simulink model "UAV_Load_Balancing_Main"  (R2025b)
settings: Solver=ode23t  StartTime=0.0  StopTime=8  FixedStep=1e-5  MaxStep=1e-5  RelTol=1e-3
libraries: nesl_utility x67, fl_lib x49, ee_lib x36
(part 2 of 2)

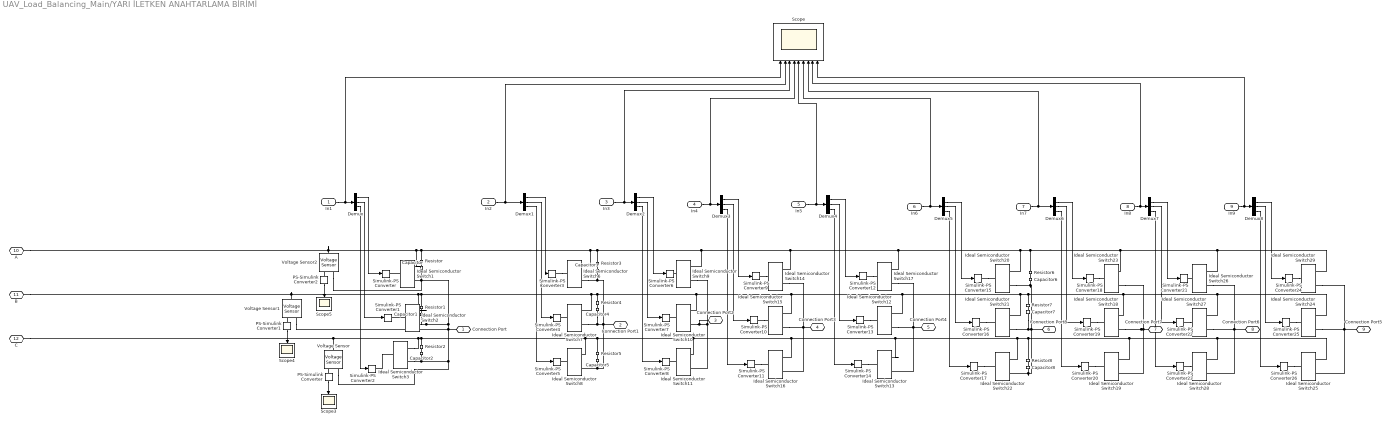
== system UAV_Load_Balancing_Main/YARI İLETKEN ANAHTARLAMA BİRİMİ ==
  In1 : Inport
  In2 : Inport  Port=2
  In3 : Inport  Port=3
  In4 : Inport  Port=4
  In5 : Inport  Port=5
  In6 : Inport  Port=6
  In7 : Inport  Port=7
  In8 : Inport  Port=8
  In9 : Inport  Port=9
  Capacitor{,3..8} (7 alike) : fl_lib/Electrical/Electrical Elements/Capacitor  c=100e-8 F  r=1e-6 Ohm  g=0 1/Ohm  i_specify=off  i_priority=None  i=0 A  i_nominal_specify=off  i_nominal_value=1  i_nominal_unit=A  v_specify=off  v_priority=None  v=0 V  v_nominal_specify=off  v_nominal_value=1  v_nominal_unit=V  vc_specify=off  vc_priority=High  vc=0 V  vc_nominal_specify=off  vc_nominal_value=1  vc_nominal_unit=V
  Capacitor1 : fl_lib/Electrical/Electrical Elements/Capacitor  c=100e-9 F  r=1e-6 Ohm  g=0 1/Ohm  i_specify=off  i_priority=None  i=0 A  i_nominal_specify=off  i_nominal_value=1  i_nominal_unit=A  v_specify=off  v_priority=None  v=0 V  v_nominal_specify=off  v_nominal_value=1  v_nominal_unit=V  vc_specify=off  vc_priority=High  vc=0 V  vc_nominal_specify=off  vc_nominal_value=1  vc_nominal_unit=V
  Capacitor2 : fl_lib/Electrical/Electrical Elements/Capacitor  c=100e-9 F  r=1e-6 Ohm  g=0 1/Ohm  i_specify=off  i_priority=None  i=0 A  i_nominal_specify=off  i_nominal_value=1  i_nominal_unit=A  v_specify=off  v_priority=None  v=0 V  v_nominal_specify=off  v_nominal_value=1  v_nominal_unit=V  vc_specify=off  vc_priority=High  vc=0 V  vc_nominal_specify=off  vc_nominal_value=1  vc_nominal_unit=V
  Demux{,1..8} (9 alike) : Demux  Outputs=3
  Ideal Semiconductor Switch{1..3,6..29} (27 alike) : ee_lib/Semiconductors & Converters/Ideal Semiconductor Switch  port_option=ee.enum.controlport.ps  Ron=0.001 Ohm  Goff=1e-6 1/Ohm  Vth=0.5 V  diode_param=ee.enum.semiconductors.protectionDiode.external  diode_Vf=0.8 V  diode_Ron=0.001 Ohm  diode_Goff=1e-5 1/Ohm  diode_C=50e-9 F  diode_iRM=-235 A  diode_iF=300 A  diode_idot=-50 A/us  diode_trr_param=ee.enum.converters.diodetrr.trr_factor  diode_trr_factor=3  diode_trr=15 us  diode_Qrr=1500 s*uA
  PS-Simulink Converter : nesl_utility/PS-Simulink Converter  PhysicalDomain=network_engine_domain  SubClassName=ps_output  LeftPortType=input  RightPortType=output  PseudoPeriodic=off  Frequencies=[]  VectorFormat=inherit  Unit=inherit  AffineConversion=off
  PS-Simulink Converter1 : nesl_utility/PS-Simulink Converter  PhysicalDomain=network_engine_domain  SubClassName=ps_output  LeftPortType=input  RightPortType=output  PseudoPeriodic=off  Frequencies=[]  VectorFormat=inherit  Unit=inherit  AffineConversion=off
  PS-Simulink Converter2 : nesl_utility/PS-Simulink Converter  PhysicalDomain=network_engine_domain  SubClassName=ps_output  LeftPortType=input  RightPortType=output  PseudoPeriodic=off  Frequencies=[]  VectorFormat=inherit  Unit=inherit  AffineConversion=off
  Resistor{,1..8} (9 alike) : fl_lib/Electrical/Electrical Elements/Resistor  R=100 Ohm  i_specify=off  i_priority=None  i=0 A  i_nominal_specify=off  i_nominal_value=1  i_nominal_unit=A  v_specify=off  v_priority=None  v=0 V  v_nominal_specify=off  v_nominal_value=1  v_nominal_unit=V
  Scope : Scope  NumInputPorts=9
      settings: ActiveDisplayYMinimum=-0.12499999999999997  ActiveDisplayYMaximum=1.125  DataLoggingVariableName=ScopeData4
  Scope3 : Scope
      settings: ActiveDisplayYMinimum=-516.00963251319388  ActiveDisplayYMaximum=519.11570917932033  DataLoggingVariableName=ScopeData9
  Scope4 : Scope
      settings: ActiveDisplayYMinimum=-401.22807276870481  ActiveDisplayYMaximum=439.38830667232617  DataLoggingVariableName=ScopeData12
  Scope5 : Scope
      settings: ActiveDisplayYMinimum=-675.65927167649568  ActiveDisplayYMaximum=614.86430923412968  DataLoggingVariableName=ScopeData13
  Simulink-PS Converter : nesl_utility/Simulink-PS Converter  PhysicalDomain=network_engine_domain  SubClassName=ps_input  LeftPortType=input  RightPortType=output  PseudoPeriodic=off  Frequencies=[]  NoiseDistribution=none  NoiseParameters=[]  Unit=V  AffineConversion=off  FilteringAndDerivatives=provide  SimscapeFilterOrder=1  InputFilterTimeConstant=0.001  UdotUserProvided=0
  Simulink-PS Converter1 : nesl_utility/Simulink-PS Converter  PhysicalDomain=network_engine_domain  SubClassName=ps_input  LeftPortType=input  RightPortType=output  PseudoPeriodic=off  Frequencies=[]  NoiseDistribution=none  NoiseParameters=[]  Unit=V  AffineConversion=off  FilteringAndDerivatives=provide  SimscapeFilterOrder=1  InputFilterTimeConstant=0.001  UdotUserProvided=0
  Simulink-PS Converter{3..26} (24 alike) : nesl_utility/Simulink-PS Converter  PhysicalDomain=network_engine_domain  SubClassName=ps_input  LeftPortType=input  RightPortType=output  PseudoPeriodic=off  Frequencies=[]  NoiseDistribution=none  NoiseParameters=[]  Unit=1  AffineConversion=off  FilteringAndDerivatives=provide  SimscapeFilterOrder=1  InputFilterTimeConstant=0.001  UdotUserProvided=0
  Simulink-PS Converter2 : nesl_utility/Simulink-PS Converter  PhysicalDomain=network_engine_domain  SubClassName=ps_input  LeftPortType=input  RightPortType=output  PseudoPeriodic=off  Frequencies=[]  NoiseDistribution=none  NoiseParameters=[]  Unit=V  AffineConversion=off  FilteringAndDerivatives=provide  SimscapeFilterOrder=1  InputFilterTimeConstant=0.001  UdotUserProvided=0
  Voltage Sensor : fl_lib/Electrical/Electrical Sensors/Voltage Sensor
  Voltage Sensor1 : fl_lib/Electrical/Electrical Sensors/Voltage Sensor
  Voltage Sensor2 : fl_lib/Electrical/Electrical Sensors/Voltage Sensor
  Connection Port : PMIOPort  Side=Right
  Connection Port1 : PMIOPort  Port=2  Side=Right
  Connection Port2 : PMIOPort  Port=3  Side=Right
  Connection Port3 : PMIOPort  Port=4  Side=Right
  Connection Port4 : PMIOPort  Port=5  Side=Right
  Connection Port8 : PMIOPort  Port=6  Side=Right
  Connection Port7 : PMIOPort  Port=7  Side=Right
  Connection Port6 : PMIOPort  Port=8  Side=Right
  Connection Port5 : PMIOPort  Port=9  Side=Right
  A : PMIOPort  Port=10  Side=Left
  B : PMIOPort  Port=11  Side=Left
  C : PMIOPort  Port=12  Side=Left
  wires:
  In1/1 -> Scope/1, Demux/1
  Demux1/3 -> Simulink-PS Converter5/1
  Demux1/1 -> Simulink-PS Converter3/1
  Demux1/2 -> Simulink-PS Converter4/1
  In2/1 -> Scope/2, Demux1/1
  Demux2/3 -> Simulink-PS Converter8/1
  Demux2/1 -> Simulink-PS Converter6/1
  Demux2/2 -> Simulink-PS Converter7/1
  In3/1 -> Scope/3, Demux2/1
  Demux3/3 -> Simulink-PS Converter11/1
  Demux3/1 -> Simulink-PS Converter9/1
  Demux3/2 -> Simulink-PS Converter10/1
  In4/1 -> Scope/4, Demux3/1
  Demux4/3 -> Simulink-PS Converter14/1
  Demux4/1 -> Simulink-PS Converter12/1
  Demux4/2 -> Simulink-PS Converter13/1
  In5/1 -> Demux4/1, Scope/5
  Demux5/3 -> Simulink-PS Converter17/1
  Demux5/1 -> Simulink-PS Converter15/1
  Demux5/2 -> Simulink-PS Converter16/1
  In6/1 -> Scope/6, Demux5/1
  Demux6/3 -> Simulink-PS Converter20/1
  Demux6/1 -> Simulink-PS Converter18/1
  Demux6/2 -> Simulink-PS Converter19/1
  In7/1 -> Scope/7, Demux6/1
  Demux7/3 -> Simulink-PS Converter23/1
  Demux7/1 -> Simulink-PS Converter21/1
  Demux7/2 -> Simulink-PS Converter22/1
  In8/1 -> Scope/8, Demux7/1
  Demux8/3 -> Simulink-PS Converter26/1
  Demux8/1 -> Simulink-PS Converter24/1
  Demux8/2 -> Simulink-PS Converter25/1
  In9/1 -> Scope/9, Demux8/1
  PS-Simulink Converter/1 -> Scope3/1
  Demux/3 -> Simulink-PS Converter2/1
  PS-Simulink Converter1/1 -> Scope4/1
  PS-Simulink Converter2/1 -> Scope5/1
  Demux/2 -> Simulink-PS Converter1/1
  Demux/1 -> Simulink-PS Converter/1
  connections:
  Connection Port/RConn1 -- Ideal Semiconductor Switch3/RConn2 -- Capacitor2/RConn1 -- Voltage Sensor/RConn2 -- Capacitor1/RConn1 -- Ideal Semiconductor Switch2/RConn2 -- Capacitor/RConn1 -- Voltage Sensor2/RConn2 -- Ideal Semiconductor Switch1/RConn2 -- Voltage Sensor1/RConn2
  B/RConn1 -- Voltage Sensor1/LConn1 -- Resistor1/LConn1 -- Ideal Semiconductor Switch7/RConn1 -- Resistor4/LConn1 -- Ideal Semiconductor Switch10/RConn1 -- Ideal Semiconductor Switch15/RConn1 -- Ideal Semiconductor Switch12/RConn1 -- Ideal Semiconductor Switch21/RConn1 -- Resistor7/LConn1 -- Ideal Semiconductor Switch18/RConn1 -- Ideal Semiconductor Switch27/RConn1 -- Ideal Semiconductor Switch24/RConn1 -- Ideal Semiconductor Switch2/RConn1
  Ideal Semiconductor Switch6/RConn2 -- Capacitor3/RConn1 -- Capacitor4/RConn1 -- Ideal Semiconductor Switch7/RConn2 -- Connection Port1/RConn1 -- Capacitor5/RConn1 -- Ideal Semiconductor Switch8/RConn2
  Ideal Semiconductor Switch29/RConn2 -- Connection Port5/RConn1 -- Ideal Semiconductor Switch24/RConn2 -- Ideal Semiconductor Switch25/RConn2
  Ideal Semiconductor Switch26/RConn2 -- Ideal Semiconductor Switch28/RConn2 -- Connection Port6/RConn1 -- Ideal Semiconductor Switch27/RConn2
  Ideal Semiconductor Switch23/RConn2 -- Ideal Semiconductor Switch18/RConn2 -- Connection Port7/RConn1 -- Ideal Semiconductor Switch19/RConn2
  Ideal Semiconductor Switch20/RConn2 -- Capacitor6/RConn1 -- Capacitor7/RConn1 -- Ideal Semiconductor Switch21/RConn2 -- Connection Port8/RConn1 -- Capacitor8/RConn1 -- Ideal Semiconductor Switch22/RConn2
  Ideal Semiconductor Switch9/RConn2 -- Connection Port2/RConn1 -- Ideal Semiconductor Switch10/RConn2 -- Ideal Semiconductor Switch11/RConn2
  Ideal Semiconductor Switch14/RConn2 -- Connection Port3/RConn1 -- Ideal Semiconductor Switch15/RConn2 -- Ideal Semiconductor Switch16/RConn2
  Ideal Semiconductor Switch17/RConn2 -- Connection Port4/RConn1 -- Ideal Semiconductor Switch12/RConn2 -- Ideal Semiconductor Switch13/RConn2
  Simulink-PS Converter4/RConn1 -- Ideal Semiconductor Switch7/LConn1
  Simulink-PS Converter3/RConn1 -- Ideal Semiconductor Switch6/LConn1
  Simulink-PS Converter5/RConn1 -- Ideal Semiconductor Switch8/LConn1
  Simulink-PS Converter6/RConn1 -- Ideal Semiconductor Switch9/LConn1
  Simulink-PS Converter7/RConn1 -- Ideal Semiconductor Switch10/LConn1
  Simulink-PS Converter8/RConn1 -- Ideal Semiconductor Switch11/LConn1
  Simulink-PS Converter9/RConn1 -- Ideal Semiconductor Switch14/LConn1
  Simulink-PS Converter10/RConn1 -- Ideal Semiconductor Switch15/LConn1
  Simulink-PS Converter11/RConn1 -- Ideal Semiconductor Switch16/LConn1
  Simulink-PS Converter12/RConn1 -- Ideal Semiconductor Switch17/LConn1
  Simulink-PS Converter13/RConn1 -- Ideal Semiconductor Switch12/LConn1
  Simulink-PS Converter14/RConn1 -- Ideal Semiconductor Switch13/LConn1
  Simulink-PS Converter15/RConn1 -- Ideal Semiconductor Switch20/LConn1
  Simulink-PS Converter16/RConn1 -- Ideal Semiconductor Switch21/LConn1
  Simulink-PS Converter17/RConn1 -- Ideal Semiconductor Switch22/LConn1
  Simulink-PS Converter18/RConn1 -- Ideal Semiconductor Switch23/LConn1
  Simulink-PS Converter19/RConn1 -- Ideal Semiconductor Switch18/LConn1
  Simulink-PS Converter20/RConn1 -- Ideal Semiconductor Switch19/LConn1
  Simulink-PS Converter21/RConn1 -- Ideal Semiconductor Switch26/LConn1
  Simulink-PS Converter22/RConn1 -- Ideal Semiconductor Switch27/LConn1
  Simulink-PS Converter23/RConn1 -- Ideal Semiconductor Switch28/LConn1
  Simulink-PS Converter24/RConn1 -- Ideal Semiconductor Switch29/LConn1
  Simulink-PS Converter25/RConn1 -- Ideal Semiconductor Switch24/LConn1
  Simulink-PS Converter26/RConn1 -- Ideal Semiconductor Switch25/LConn1
  A/RConn1 -- Voltage Sensor2/LConn1 -- Resistor/LConn1 -- Ideal Semiconductor Switch6/RConn1 -- Resistor3/LConn1 -- Ideal Semiconductor Switch9/RConn1 -- Ideal Semiconductor Switch14/RConn1 -- Resistor6/LConn1 -- Ideal Semiconductor Switch23/RConn1 -- Ideal Semiconductor Switch26/RConn1 -- Ideal Semiconductor Switch29/RConn1 -- Ideal Semiconductor Switch20/RConn1 -- Ideal Semiconductor Switch17/RConn1 -- Ideal Semiconductor Switch1/RConn1
  PS-Simulink Converter/LConn1 -- Voltage Sensor/RConn1
  Ideal Semiconductor Switch19/RConn1 -- Resistor8/LConn1 -- Resistor5/LConn1 -- Voltage Sensor/LConn1 -- C/RConn1 -- Ideal Semiconductor Switch3/RConn1 -- Resistor2/LConn1 -- Ideal Semiconductor Switch8/RConn1 -- Ideal Semiconductor Switch11/RConn1 -- Ideal Semiconductor Switch16/RConn1 -- Ideal Semiconductor Switch13/RConn1 -- Ideal Semiconductor Switch22/RConn1 -- Ideal Semiconductor Switch28/RConn1 -- Ideal Semiconductor Switch25/RConn1
  PS-Simulink Converter1/LConn1 -- Voltage Sensor1/RConn1
  PS-Simulink Converter2/LConn1 -- Voltage Sensor2/RConn1
  Ideal Semiconductor Switch1/LConn1 -- Simulink-PS Converter/RConn1
  Ideal Semiconductor Switch2/LConn1 -- Simulink-PS Converter1/RConn1
  Ideal Semiconductor Switch3/LConn1 -- Simulink-PS Converter2/RConn1
  Resistor/RConn1 -- Capacitor/LConn1
  Resistor1/RConn1 -- Capacitor1/LConn1
  Resistor2/RConn1 -- Capacitor2/LConn1
  Resistor3/RConn1 -- Capacitor3/LConn1
  Resistor4/RConn1 -- Capacitor4/LConn1
  Resistor5/RConn1 -- Capacitor5/LConn1
  Resistor6/RConn1 -- Capacitor6/LConn1
  Resistor7/RConn1 -- Capacitor7/LConn1
  Resistor8/RConn1 -- Capacitor8/LConn1

== matlab function UAV_Load_Balancing_Main/RMS Calculation Block/MATLAB Function1 ==
  data: IA input; IrmsA output; IB input; IC input; IrmsB output; IrmsC output
function [IrmsA, IrmsB, IrmsC] = PhaseRMS(IA, IB, IC)

% Sistem frekansı: 400 Hz
% Örnekleme zamanı: 10 us
% Bir periyot: 2.5 ms
% Örnek sayısı: 250

N = 250;

persistent BufA BufB BufC
persistent Index SumA SumB SumC
persistent RMS_A RMS_B RMS_C

if isempty(Index)

    BufA = zeros(N,1);
    BufB = zeros(N,1);
    BufC = zeros(N,1);

    Index = 1;

    SumA = 0;
    SumB = 0;
    SumC = 0;

    RMS_A = 0;
    RMS_B = 0;
    RMS_C = 0;

end

% Önceki örneklerin karelerini çıkar
SumA = SumA - BufA(Index)^2;
SumB = SumB - BufB(Index)^2;
SumC = SumC - BufC(Index)^2;

% Yeni örnekleri kaydet
BufA(Index) = IA;
BufB(Index) = IB;
BufC(Index) = IC;

% Kareler toplamını güncelle
SumA = SumA + IA^2;
SumB = SumB + IB^2;
SumC = SumC + IC^2;

% Bir periyot tamamlanınca RMS değerlerini güncelle
if Index == N

    RMS_A = sqrt(max(SumA,0)/N);
    RMS_B = sqrt(max(SumB,0)/N);
    RMS_C = sqrt(max(SumC,0)/N);

end

% Son tamamlanmış RMS değerlerini çıkışa ver
IrmsA = RMS_A;
IrmsB = RMS_B;
IrmsC = RMS_C;

% Örnek indeksini ilerlet
Index = Index + 1;

if Index > N
    Index = 1;
end

end

== matlab function UAV_Load_Balancing_Main/MATLAB Function ==
  settings: updateMethod=DISCRETE  sampleTime=0.001
  data: Iphase input; Iload input; Enable input; Reset input; t input; SwitchCmd output; FDI output

function [SwitchCmd, FDI] = LoadBalancing(Iphase, Iload, Enable, Reset, t)

% Iphase: 3x1 faz RMS akimlari [A; B; C]
% Iload:  9x1 yuk RMS akimlari
% Enable: algoritma etkinlestirme girisi
% Reset:  baslangic/reset girisi
% t:      Clock blogundan gelen zaman (s)
% SwitchCmd: 27x1 anahtar komutlari
% FDI: faz dengesizlik indeksi (%)

StartDelay = 0.35;
MoveDelay  = 0.1;
FDI_Start  = 5.0;
FDI_Stop   = 3.0;

persistent LoadPhase LastMoveTime Balancing

% Baslangic dagilimi: 1=A, 2=B, 3=C
if isempty(LoadPhase) || Reset ~= 0
    LoadPhase = [1; 2; 1; 3; 2; 1; 3; 2; 3];
    LastMoveTime = -1e6;
    Balancing = false;
end

% FDI hesapla
Iavg = mean(Iphase);

if Iavg > 0
    FDI = max(abs(Iphase - Iavg)) / Iavg * 100;
else
    FDI = 0;
end

% Mevcut dagilima gore anahtarlari olustur
SwitchCmd = zeros(27,1);

for k = 1:9
    idx = (k-1)*3 + LoadPhase(k);
    SwitchCmd(idx) = 1;
end

% Reset aktifse mevcut baslangic komutlarini ver
if Reset ~= 0
    return;
end

% Enable kapaliysa aktarim yapma
if Enable == 0
    return;
end

% Baslangicta 0.35 saniye bekle
if t < StartDelay
    return;
end

% FDI histerezisi
if FDI > FDI_Start
    Balancing = true;
elseif FDI <= FDI_Stop
    Balancing = false;
end

% Dengeleme gerekmiyorsa cik
if ~Balancing
    return;
end

% Aktarimlar arasinda 50 ms bekle
if (t - LastMoveTime) < MoveDelay
    return;
end

% En yuklu ve en az yuklu fazlari bul
[~, SourcePhase] = max(Iphase);
[~, TargetPhase] = min(Iphase);

% En yuklu fazdaki en kucuk akimli yuku bul
SelectedLoad = 0;
SmallestCurrent = inf;

for k = 1:9
    if LoadPhase(k) == SourcePhase && Iload(k) < SmallestCurrent
        SmallestCurrent = Iload(k);
        SelectedLoad = k;
    end
end

% Kaynak fazda uygun yuk yoksa aktarim yapma
if SelectedLoad == 0
    return;
end

% Secilen yuku hedef faza aktar
LoadPhase(SelectedLoad) = TargetPhase;
LastMoveTime = t;

% Yeni anahtar komutlarini olustur
SwitchCmd = zeros(27,1);

for k = 1:9
    idx = (k-1)*3 + LoadPhase(k);
    SwitchCmd(idx) = 1;
end

end

== stateflow chart UAV_Load_Balancing_Main/Load Chart/Chart ==
  state G5
    during:
    Phase = 1;
  state G6
    during:
    Phase = 2
    ;
  state G7
    during:
    Phase = 3
    ;
  state G9
    during:
    Phase = 4
    ;
  (default) -> G5
  G7 -> G9 : [after(1.8,sec)
      | ]
  G6 -> G7 : [after(2,sec)
      | ]
  G5 -> G6 : [after(1.8,sec)
      | ]
  data: Phase output

== matlab function UAV_Load_Balancing_Main/Load Chart/MATLAB Function2 ==
  data: Phase input; S output; PF output

function [S, PF] = fcn(Phase)

S = zeros(1,9);
PF = zeros(1,9);

if Phase == 1
    S  = [1150 1900 5891 438 2657 400 480 4000 5400];
    PF = [0.60 0.94 0.95 0.85 0.60 1.00 1.00 0.60 0.92];

elseif Phase == 2
    S  = [1150 4200 5891 438 2657 750 480 4000 5400];
    PF = [0.60 0.97 0.95 0.85 0.60 1.00 1.00 0.60 0.92];

elseif Phase == 3
    S  = [1150 4200 6621 438 2657 400 480 4000 5400];
    PF = [0.60 0.97 0.97 0.85 0.60 1.00 1.00 0.60 0.92];

elseif Phase == 4
    S  = [1150 4200 5891 438 2657 400 480 4000 5400];
    PF = [0.60 0.97 0.95 0.85 0.60 1.00 1.00 0.60 0.92];
end

end

== matlab function UAV_Load_Balancing_Main/Load Chart/MATLAB Function3 ==
  data: S input; R output; PF input; L output

function [R, L] = CalculateRL(S, PF)

V = 115;       % RMS gerilim (V)
f = 400;       % Frekans (Hz)
w = 2*pi*f;

% Aktif ve reaktif guc
P = S .* PF;
Q = S .* sqrt(max(0, 1 - PF.^2));

% Direnc ve enduktans
R = zeros(size(S));
L = zeros(size(S));

idx = S > 0;

R(idx) = V^2 .* P(idx) ./ S(idx).^2;

idxL = S > 0 & Q > 0;

L(idxL) = V^2 .* Q(idxL) ./ ...
          (w .* S(idxL).^2);

end

function [P,Q] = fcn(S,PF)

P = S .* PF;
Q = S .* sqrt(1 - PF.^2);

end

== matlab function UAV_Load_Balancing_Main/RMS Calculation Block 2/MATLAB Function2 ==
  settings: updateMethod=DISCRETE
  data: I1 input; Irms1 output; I2 input; I3 input; I4 input; I5 input; I6 input; I7 input; I8 input; I9 input; Irms2 output; Irms3 output; Irms4 output; Irms5 output; Irms6 output; Irms7 output; Irms8 output; Irms9 output
function [Irms1, Irms2, Irms3, Irms4, Irms5, ...
          Irms6, Irms7, Irms8, Irms9] = LoadRMS( ...
          I1, I2, I3, I4, I5, I6, I7, I8, I9)

N = 250;

persistent Buffer SumSq Index
persistent RMS

if isempty(Index)
    Buffer = zeros(N,9);
    SumSq = zeros(1,9);
    Index = 1;
    RMS = zeros(1,9);
end

% Anlik akimlari vektore al
I = [I1 I2 I3 I4 I5 I6 I7 I8 I9];

% Eski ornegin karesini cikar
SumSq = SumSq - Buffer(Index,:).^2;

% Yeni ornegi kaydet
Buffer(Index,:) = I;

% Kareler toplamini guncelle
SumSq = SumSq + I.^2;

% Tam bir periyot tamamlandi mi?
if Index == N
    RMS = sqrt(max(SumSq,0)/N);
end

% Dokuz RMS cikisi
Irms1 = RMS(1);
Irms2 = RMS(2);
Irms3 = RMS(3);
Irms4 = RMS(4);
Irms5 = RMS(5);
Irms6 = RMS(6);
Irms7 = RMS(7);
Irms8 = RMS(8);
Irms9 = RMS(9);

% Sonraki ornek
Index = Index + 1;

if Index > N
    Index = 1;
end

end

== matlab function UAV_Load_Balancing_Main/RMS Calculation Block/MATLAB Function ==
  data: Iphase input; FDI output
function FDI = FDI_Calculation(Iphase)
% Iphase: [IrmsA; IrmsB; IrmsC] seklinde 3x1 kaynak RMS akimlari

% 1. Uc fazin ortalama akimini hesapla
Iavg = (Iphase(1) + Iphase(2) + Iphase(3)) / 3;

% 2. Sıfıra bölme hatasını önleyerek FDI yüzde (%) değerini çıkar
if Iavg > 0
    % Ortalamadan olan maksimum sapmayi bul ve yüzdeye cevir
    FDI = max(abs(Iphase - Iavg)) / Iavg * 100;
else
    FDI = 0;
end

end
